simulink model "IEEE33_TR_TEMPORAL_RECOGNIZABILITY_MASTER"  (R2026b)
settings: Solver=ode23t  StopTime=0.2  MaxStep=1e-5
undefined symbols (not defined in the file): Three_PhaseBreaker_class, Three_PhaseSeriesRLCLoad_class, Three_PhaseSource_class, Three_PhaseV_IMeasuremen_class
libraries: ee_lib x146, nesl_utility x106, fl_lib x33, eeRmsMeasurement x2
(part 2 of 7)

== system IEEE33_TR_TEMPORAL_RECOGNIZABILITY_MASTER/Bus_22 ==
  Bus Load 22 : Subsystem
      settings: AttributesFormatString=\n  OpenFcn=elec.conv.unmask(gcb);
  Bus_22 : Subsystem
      settings: OpenFcn=elec.conv.unmask(gcb);
  CB3-2 : Subsystem
      settings: OpenFcn=elec.conv.unmask(gcb);
  VI Recorder3 : Subsystem
  InPhaseA : PMIOPort  Side=Left
  InPhaseB : PMIOPort  Port=2  Side=Left
  InPhaseC : PMIOPort  Port=3  Side=Left
  OutPhaseA : PMIOPort  Port=4  Side=Right
  OutPhaseB : PMIOPort  Port=5  Side=Right
  OutPhaseC : PMIOPort  Port=6  Side=Right
  wires:
  [CB22to12] -> CB3-2/1(com)
  Bus_22/2(Iabc) -> VI Recorder3/2(Irec)
  Bus_22/1(Vabc) -> VI Recorder3/1(Vrec)
  connections:
  CB3-2/RConn3 -- OutPhaseC/RConn1
  Bus_22/RConn2 -- Bus Load 22/LConn2 -- CB3-2/LConn2
  Bus_22/RConn3 -- Bus Load 22/LConn3 -- CB3-2/LConn3
  CB3-2/RConn1 -- OutPhaseA/RConn1
  CB3-2/RConn2 -- OutPhaseB/RConn1
  Bus Load 22/LConn1 -- CB3-2/LConn1 -- Bus_22/RConn1
  InPhaseA/RConn1 -- Bus_22/LConn1
  InPhaseB/RConn1 -- Bus_22/LConn2
  InPhaseC/RConn1 -- Bus_22/LConn3

== system IEEE33_TR_TEMPORAL_RECOGNIZABILITY_MASTER/Bus_23 ==
  Bus Load 23 : Subsystem
      settings: AttributesFormatString=\n  OpenFcn=elec.conv.unmask(gcb);
  Bus_23 : Subsystem
      settings: OpenFcn=elec.conv.unmask(gcb);
  CB3-2 : Subsystem
      settings: OpenFcn=elec.conv.unmask(gcb);
  VI Recorder32 : Subsystem
  InPhaseA : PMIOPort  Side=Left
  InPhaseB : PMIOPort  Port=2  Side=Left
  InPhaseC : PMIOPort  Port=3  Side=Left
  OutPhaseA : PMIOPort  Port=4  Side=Right
  OutPhaseB : PMIOPort  Port=5  Side=Right
  OutPhaseC : PMIOPort  Port=6  Side=Right
  wires:
  Bus_23/2(Iabc) -> VI Recorder32/2(Irec)
  Bus_23/1(Vabc) -> VI Recorder32/1(Vrec)
  [CB23to24] -> CB3-2/1(com)
  connections:
  Bus_23/RConn1 -- CB3-2/LConn1 -- Bus Load 23/LConn1
  CB3-2/RConn3 -- OutPhaseC/RConn1
  Bus Load 23/LConn2 -- CB3-2/LConn2 -- Bus_23/RConn2
  Bus Load 23/LConn3 -- CB3-2/LConn3 -- Bus_23/RConn3
  CB3-2/RConn1 -- OutPhaseA/RConn1
  CB3-2/RConn2 -- OutPhaseB/RConn1
  InPhaseA/RConn1 -- Bus_23/LConn1
  InPhaseB/RConn1 -- Bus_23/LConn2
  InPhaseC/RConn1 -- Bus_23/LConn3

== system IEEE33_TR_TEMPORAL_RECOGNIZABILITY_MASTER/Bus_24 ==
  Bus Load 24 : Subsystem
      settings: AttributesFormatString=\n  OpenFcn=elec.conv.unmask(gcb);
  Bus_24 : Subsystem
      settings: OpenFcn=elec.conv.unmask(gcb);
  CB3-2 : Subsystem
      settings: OpenFcn=elec.conv.unmask(gcb);
  VI Recorder31 : Subsystem
  InPhaseA : PMIOPort  Side=Left
  InPhaseB : PMIOPort  Port=2  Side=Left
  InPhaseC : PMIOPort  Port=3  Side=Left
  OutPhaseA : PMIOPort  Port=4  Side=Right
  OutPhaseB : PMIOPort  Port=5  Side=Right
  OutPhaseC : PMIOPort  Port=6  Side=Right
  wires:
  Bus_24/1(Vabc) -> VI Recorder31/1(Vrec)
  Bus_24/2(Iabc) -> VI Recorder31/2(Irec)
  [CB24to25] -> CB3-2/1(com)
  connections:
  Bus_24/RConn1 -- CB3-2/LConn1 -- Bus Load 24/LConn1
  CB3-2/RConn3 -- OutPhaseC/RConn1
  Bus Load 24/LConn2 -- CB3-2/LConn2 -- Bus_24/RConn2
  Bus Load 24/LConn3 -- CB3-2/LConn3 -- Bus_24/RConn3
  CB3-2/RConn1 -- OutPhaseA/RConn1
  CB3-2/RConn2 -- OutPhaseB/RConn1
  InPhaseA/RConn1 -- Bus_24/LConn1
  InPhaseB/RConn1 -- Bus_24/LConn2
  InPhaseC/RConn1 -- Bus_24/LConn3

== system IEEE33_TR_TEMPORAL_RECOGNIZABILITY_MASTER/Bus_25 ==
  Bus Load 25 : Subsystem
      settings: AttributesFormatString=\n  OpenFcn=elec.conv.unmask(gcb);
  Bus_25 : Subsystem
      settings: OpenFcn=elec.conv.unmask(gcb);
  CB3-2 : Subsystem
      settings: OpenFcn=elec.conv.unmask(gcb);
  VI Recorder30 : Subsystem
  InPhaseA : PMIOPort  Side=Left
  InPhaseB : PMIOPort  Port=2  Side=Left
  InPhaseC : PMIOPort  Port=3  Side=Left
  OutPhaseA : PMIOPort  Port=4  Side=Right
  OutPhaseB : PMIOPort  Port=5  Side=Right
  OutPhaseC : PMIOPort  Port=6  Side=Right
  wires:
  Bus_25/2(Iabc) -> VI Recorder30/2(Irec)
  Bus_25/1(Vabc) -> VI Recorder30/1(Vrec)
  [CB25to29] -> CB3-2/1(com)
  connections:
  Bus_25/RConn1 -- CB3-2/LConn1 -- Bus Load 25/LConn1
  CB3-2/RConn3 -- OutPhaseC/RConn1
  Bus Load 25/LConn2 -- CB3-2/LConn2 -- Bus_25/RConn2
  Bus_25/RConn3 -- CB3-2/LConn3 -- Bus Load 25/LConn3
  CB3-2/RConn1 -- OutPhaseA/RConn1
  CB3-2/RConn2 -- OutPhaseB/RConn1
  InPhaseB/RConn1 -- Bus_25/LConn2
  InPhaseA/RConn1 -- Bus_25/LConn1
  InPhaseC/RConn1 -- Bus_25/LConn3

== system IEEE33_TR_TEMPORAL_RECOGNIZABILITY_MASTER/Bus_26 ==
  Bus Load 26 : Subsystem
      settings: AttributesFormatString=\n  OpenFcn=elec.conv.unmask(gcb);
  Bus_26 : Subsystem
      settings: OpenFcn=elec.conv.unmask(gcb);
  CB3-2 : Subsystem
      settings: OpenFcn=elec.conv.unmask(gcb);
  VI Recorder22 : Subsystem
  InPhaseA : PMIOPort  Side=Left
  InPhaseB : PMIOPort  Port=2  Side=Left
  InPhaseC : PMIOPort  Port=3  Side=Left
  OutPhaseA : PMIOPort  Port=4  Side=Right
  OutPhaseB : PMIOPort  Port=5  Side=Right
  OutPhaseC : PMIOPort  Port=6  Side=Right
  wires:
  Bus_26/2(Iabc) -> VI Recorder22/2(Irec)
  Bus_26/1(Vabc) -> VI Recorder22/1(Vrec)
  [CB26to27] -> CB3-2/1(com)
  connections:
  CB3-2/RConn3 -- OutPhaseC/RConn1
  Bus Load 26/LConn2 -- CB3-2/LConn2 -- Bus_26/RConn2
  Bus_26/RConn3 -- CB3-2/LConn3 -- Bus Load 26/LConn3
  CB3-2/RConn1 -- OutPhaseA/RConn1
  CB3-2/RConn2 -- OutPhaseB/RConn1
  Bus_26/RConn1 -- CB3-2/LConn1 -- Bus Load 26/LConn1
  InPhaseA/RConn1 -- Bus_26/LConn1
  InPhaseB/RConn1 -- Bus_26/LConn2
  InPhaseC/RConn1 -- Bus_26/LConn3

== system IEEE33_TR_TEMPORAL_RECOGNIZABILITY_MASTER/Bus_27 ==
  Bus Load 27 : Subsystem
      settings: AttributesFormatString=\n  OpenFcn=elec.conv.unmask(gcb);
  Bus_27 : Subsystem
      settings: OpenFcn=elec.conv.unmask(gcb);
  CB3-2 : Subsystem
      settings: OpenFcn=elec.conv.unmask(gcb);
  VI Recorder23 : Subsystem
  InPhaseA : PMIOPort  Side=Left
  InPhaseB : PMIOPort  Port=2  Side=Left
  InPhaseC : PMIOPort  Port=3  Side=Left
  OutPhaseA : PMIOPort  Port=4  Side=Right
  OutPhaseB : PMIOPort  Port=5  Side=Right
  OutPhaseC : PMIOPort  Port=6  Side=Right
  wires:
  Bus_27/1(Vabc) -> VI Recorder23/1(Vrec)
  Bus_27/2(Iabc) -> VI Recorder23/2(Irec)
  [CB27to28] -> CB3-2/1(com)
  connections:
  CB3-2/LConn1 -- Bus Load 27/LConn1 -- Bus_27/RConn1
  CB3-2/RConn3 -- OutPhaseC/RConn1
  CB3-2/LConn2 -- Bus Load 27/LConn2 -- Bus_27/RConn2
  Bus_27/RConn3 -- Bus Load 27/LConn3 -- CB3-2/LConn3
  CB3-2/RConn1 -- OutPhaseA/RConn1
  CB3-2/RConn2 -- OutPhaseB/RConn1
  InPhaseA/RConn1 -- Bus_27/LConn1
  InPhaseB/RConn1 -- Bus_27/LConn2
  InPhaseC/RConn1 -- Bus_27/LConn3

== system IEEE33_TR_TEMPORAL_RECOGNIZABILITY_MASTER/Bus_28 ==
  Bus Load 28 : Subsystem
      settings: AttributesFormatString=\n  OpenFcn=elec.conv.unmask(gcb);
  Bus_28 : Subsystem
      settings: OpenFcn=elec.conv.unmask(gcb);
  CB3-2 : Subsystem
      settings: OpenFcn=elec.conv.unmask(gcb);
  VI Recorder24 : Subsystem
  InPhaseA : PMIOPort  Side=Left
  InPhaseB : PMIOPort  Port=2  Side=Left
  InPhaseC : PMIOPort  Port=3  Side=Left
  OutPhaseA : PMIOPort  Port=4  Side=Right
  OutPhaseB : PMIOPort  Port=5  Side=Right
  OutPhaseC : PMIOPort  Port=6  Side=Right
  wires:
  Bus_28/2(Iabc) -> VI Recorder24/2(Irec)
  Bus_28/1(Vabc) -> VI Recorder24/1(Vrec)
  [CB28to29] -> CB3-2/1(com)
  connections:
  Bus Load 28/LConn1 -- CB3-2/LConn1 -- Bus_28/RConn1
  CB3-2/RConn3 -- OutPhaseC/RConn1
  Bus Load 28/LConn2 -- CB3-2/LConn2 -- Bus_28/RConn2
  Bus Load 28/LConn3 -- CB3-2/LConn3 -- Bus_28/RConn3
  CB3-2/RConn1 -- OutPhaseA/RConn1
  CB3-2/RConn2 -- OutPhaseB/RConn1
  InPhaseA/RConn1 -- Bus_28/LConn1
  InPhaseB/RConn1 -- Bus_28/LConn2
  InPhaseC/RConn1 -- Bus_28/LConn3

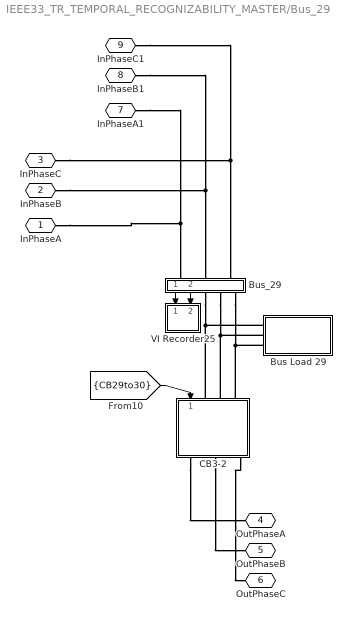
== system IEEE33_TR_TEMPORAL_RECOGNIZABILITY_MASTER/Bus_29 ==
  Bus Load 29 : Subsystem
      settings: AttributesFormatString=\n  OpenFcn=elec.conv.unmask(gcb);
  Bus_29 : Subsystem
      settings: OpenFcn=elec.conv.unmask(gcb);
  CB3-2 : Subsystem
      settings: OpenFcn=elec.conv.unmask(gcb);
  VI Recorder25 : Subsystem
  InPhaseA : PMIOPort  Side=Left
  InPhaseB : PMIOPort  Port=2  Side=Left
  InPhaseC : PMIOPort  Port=3  Side=Left
  OutPhaseA : PMIOPort  Port=4  Side=Right
  OutPhaseB : PMIOPort  Port=5  Side=Right
  OutPhaseC : PMIOPort  Port=6  Side=Right
  InPhaseA1 : PMIOPort  Port=7  Side=Left
  InPhaseB1 : PMIOPort  Port=8  Side=Left
  InPhaseC1 : PMIOPort  Port=9  Side=Left
  wires:
  Bus_29/1(Vabc) -> VI Recorder25/1(Vrec)
  Bus_29/2(Iabc) -> VI Recorder25/2(Irec)
  [CB29to30] -> CB3-2/1(com)
  connections:
  Bus_29/RConn1 -- CB3-2/LConn1 -- Bus Load 29/LConn1
  CB3-2/RConn3 -- OutPhaseC/RConn1
  Bus Load 29/LConn2 -- CB3-2/LConn2 -- Bus_29/RConn2
  Bus Load 29/LConn3 -- CB3-2/LConn3 -- Bus_29/RConn3
  CB3-2/RConn1 -- OutPhaseA/RConn1
  CB3-2/RConn2 -- OutPhaseB/RConn1
  InPhaseB1/RConn1 -- InPhaseB/RConn1 -- Bus_29/LConn2
  InPhaseA1/RConn1 -- InPhaseA/RConn1 -- Bus_29/LConn1
  InPhaseC1/RConn1 -- InPhaseC/RConn1 -- Bus_29/LConn3

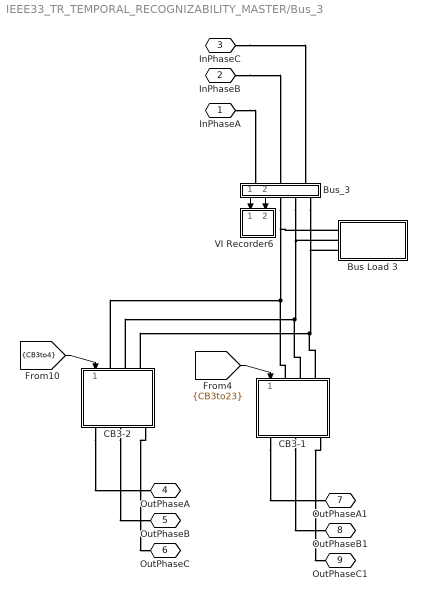
== system IEEE33_TR_TEMPORAL_RECOGNIZABILITY_MASTER/Bus_3 ==
  Bus Load 3 : Subsystem
      settings: AttributesFormatString=\n  OpenFcn=elec.conv.unmask(gcb);
  Bus_3 : Subsystem
      settings: OpenFcn=elec.conv.unmask(gcb);
  CB3-1 : Subsystem
      settings: OpenFcn=elec.conv.unmask(gcb);
  CB3-2 : Subsystem
      settings: OpenFcn=elec.conv.unmask(gcb);
  VI Recorder6 : Subsystem
  InPhaseA : PMIOPort  Side=Left
  InPhaseB : PMIOPort  Port=2  Side=Left
  InPhaseC : PMIOPort  Port=3  Side=Left
  OutPhaseA : PMIOPort  Port=4  Side=Right
  OutPhaseB : PMIOPort  Port=5  Side=Right
  OutPhaseC : PMIOPort  Port=6  Side=Right
  OutPhaseA1 : PMIOPort  Port=7  Side=Right
  OutPhaseB1 : PMIOPort  Port=8  Side=Right
  OutPhaseC1 : PMIOPort  Port=9  Side=Right
  wires:
  Bus_3/2(Iabc) -> VI Recorder6/2(Irec)
  Bus_3/1(Vabc) -> VI Recorder6/1(Vrec)
  [CB3to4] -> CB3-2/1(com)
  [CB3to23] -> CB3-1/1(com)
  connections:
  CB3-2/LConn1 -- CB3-1/LConn1 -- Bus Load 3/LConn1 -- Bus_3/RConn1
  CB3-2/RConn3 -- OutPhaseC/RConn1
  CB3-1/LConn2 -- Bus Load 3/LConn2 -- Bus_3/RConn2 -- CB3-2/LConn2
  CB3-1/LConn3 -- Bus_3/RConn3 -- Bus Load 3/LConn3 -- CB3-2/LConn3
  CB3-2/RConn1 -- OutPhaseA/RConn1
  CB3-2/RConn2 -- OutPhaseB/RConn1
  CB3-1/RConn3 -- OutPhaseC1/RConn1
  CB3-1/RConn1 -- OutPhaseA1/RConn1
  CB3-1/RConn2 -- OutPhaseB1/RConn1
  InPhaseA/RConn1 -- Bus_3/LConn1
  InPhaseB/RConn1 -- Bus_3/LConn2
  InPhaseC/RConn1 -- Bus_3/LConn3

== system IEEE33_TR_TEMPORAL_RECOGNIZABILITY_MASTER/Bus_30 ==
  Bus Load 30 : Subsystem
      settings: AttributesFormatString=\n  OpenFcn=elec.conv.unmask(gcb);
  Bus_30 : Subsystem
      settings: OpenFcn=elec.conv.unmask(gcb);
  CB3-2 : Subsystem
      settings: OpenFcn=elec.conv.unmask(gcb);
  VI Recorder26 : Subsystem
  InPhaseA : PMIOPort  Side=Left
  InPhaseB : PMIOPort  Port=2  Side=Left
  InPhaseC : PMIOPort  Port=3  Side=Left
  OutPhaseA : PMIOPort  Port=4  Side=Right
  OutPhaseB : PMIOPort  Port=5  Side=Right
  OutPhaseC : PMIOPort  Port=6  Side=Right
  wires:
  Bus_30/1(Vabc) -> VI Recorder26/1(Vrec)
  Bus_30/2(Iabc) -> VI Recorder26/2(Irec)
  [CB30to31] -> CB3-2/1(com)
  connections:
  Bus_30/RConn1 -- CB3-2/LConn1 -- Bus Load 30/LConn1
  CB3-2/RConn3 -- OutPhaseC/RConn1
  Bus Load 30/LConn2 -- CB3-2/LConn2 -- Bus_30/RConn2
  Bus Load 30/LConn3 -- CB3-2/LConn3 -- Bus_30/RConn3
  CB3-2/RConn1 -- OutPhaseA/RConn1
  CB3-2/RConn2 -- OutPhaseB/RConn1
  InPhaseB/RConn1 -- Bus_30/LConn2
  InPhaseA/RConn1 -- Bus_30/LConn1
  InPhaseC/RConn1 -- Bus_30/LConn3

== system IEEE33_TR_TEMPORAL_RECOGNIZABILITY_MASTER/Bus_31 ==
  Bus Load 31 : Subsystem
      settings: AttributesFormatString=\n  OpenFcn=elec.conv.unmask(gcb);
  Bus_31 : Subsystem
      settings: OpenFcn=elec.conv.unmask(gcb);
  CB3-2 : Subsystem
      settings: OpenFcn=elec.conv.unmask(gcb);
  VI Recorder27 : Subsystem
  InPhaseA : PMIOPort  Side=Left
  InPhaseB : PMIOPort  Port=2  Side=Left
  InPhaseC : PMIOPort  Port=3  Side=Left
  OutPhaseA : PMIOPort  Port=4  Side=Right
  OutPhaseB : PMIOPort  Port=5  Side=Right
  OutPhaseC : PMIOPort  Port=6  Side=Right
  wires:
  Bus_31/2(Iabc) -> VI Recorder27/2(Irec)
  Bus_31/1(Vabc) -> VI Recorder27/1(Vrec)
  [CB31to32] -> CB3-2/1(com)
  connections:
  Bus_31/RConn1 -- CB3-2/LConn1 -- Bus Load 31/LConn1
  CB3-2/RConn3 -- OutPhaseC/RConn1
  Bus Load 31/LConn2 -- CB3-2/LConn2 -- Bus_31/RConn2
  Bus Load 31/LConn3 -- CB3-2/LConn3 -- Bus_31/RConn3
  CB3-2/RConn1 -- OutPhaseA/RConn1
  CB3-2/RConn2 -- OutPhaseB/RConn1
  InPhaseA/RConn1 -- Bus_31/LConn1
  Bus_31/LConn2 -- InPhaseB/RConn1
  InPhaseC/RConn1 -- Bus_31/LConn3

== system IEEE33_TR_TEMPORAL_RECOGNIZABILITY_MASTER/Bus_32 ==
  Bus Load 32 : Subsystem
      settings: AttributesFormatString=\n  OpenFcn=elec.conv.unmask(gcb);
  Bus_32 : Subsystem
      settings: OpenFcn=elec.conv.unmask(gcb);
  CB3-2 : Subsystem
      settings: OpenFcn=elec.conv.unmask(gcb);
  VI Recorder28 : Subsystem
  InPhaseA : PMIOPort  Side=Left
  InPhaseB : PMIOPort  Port=2  Side=Left
  InPhaseC : PMIOPort  Port=3  Side=Left
  OutPhaseA : PMIOPort  Port=4  Side=Right
  OutPhaseB : PMIOPort  Port=5  Side=Right
  OutPhaseC : PMIOPort  Port=6  Side=Right
  wires:
  Bus_32/2(Iabc) -> VI Recorder28/2(Irec)
  Bus_32/1(Vabc) -> VI Recorder28/1(Vrec)
  [CB32to33] -> CB3-2/1(com)
  connections:
  Bus_32/RConn1 -- CB3-2/LConn1 -- Bus Load 32/LConn1
  CB3-2/RConn3 -- OutPhaseC/RConn1
  Bus Load 32/LConn2 -- CB3-2/LConn2 -- Bus_32/RConn2
  Bus_32/RConn3 -- Bus Load 32/LConn3 -- CB3-2/LConn3
  CB3-2/RConn1 -- OutPhaseA/RConn1
  CB3-2/RConn2 -- OutPhaseB/RConn1
  InPhaseA/RConn1 -- Bus_32/LConn1
  InPhaseB/RConn1 -- Bus_32/LConn2
  InPhaseC/RConn1 -- Bus_32/LConn3

== system IEEE33_TR_TEMPORAL_RECOGNIZABILITY_MASTER/Bus_33 ==
  Bus Load 33 : Subsystem
      settings: AttributesFormatString=\n  OpenFcn=elec.conv.unmask(gcb);
  Bus_33 : Subsystem
      settings: OpenFcn=elec.conv.unmask(gcb);
  VI Recorder29 : Subsystem
  InPhaseA : PMIOPort  Side=Left
  InPhaseB : PMIOPort  Port=2  Side=Left
  InPhaseC : PMIOPort  Port=3  Side=Left
  OutPhaseA : PMIOPort  Port=4  Side=Right
  OutPhaseB : PMIOPort  Port=5  Side=Right
  OutPhaseC : PMIOPort  Port=6  Side=Right
  wires:
  Bus_33/2(Iabc) -> VI Recorder29/2(Irec)
  Bus_33/1(Vabc) -> VI Recorder29/1(Vrec)
  connections:
  Bus Load 33/LConn1 -- Bus_33/RConn1 -- OutPhaseA/RConn1
  Bus Load 33/LConn2 -- OutPhaseB/RConn1 -- Bus_33/RConn2
  Bus_33/RConn3 -- OutPhaseC/RConn1 -- Bus Load 33/LConn3
  InPhaseA/RConn1 -- Bus_33/LConn1
  InPhaseB/RConn1 -- Bus_33/LConn2
  InPhaseC/RConn1 -- Bus_33/LConn3

== system IEEE33_TR_TEMPORAL_RECOGNIZABILITY_MASTER/Bus_4 ==
  Bus Load 4 : Subsystem
      settings: AttributesFormatString=\n  OpenFcn=elec.conv.unmask(gcb);
  Bus_4 : Subsystem
      settings: OpenFcn=elec.conv.unmask(gcb);
  CB3-2 : Subsystem
      settings: OpenFcn=elec.conv.unmask(gcb);
  VI Recorder7 : Subsystem
  InPhaseA : PMIOPort  Side=Left
  InPhaseB : PMIOPort  Port=2  Side=Left
  InPhaseC : PMIOPort  Port=3  Side=Left
  OutPhaseA : PMIOPort  Port=4  Side=Right
  OutPhaseB : PMIOPort  Port=5  Side=Right
  OutPhaseC : PMIOPort  Port=6  Side=Right
  wires:
  Bus_4/1(Vabc) -> VI Recorder7/1(Vrec)
  Bus_4/2(Iabc) -> VI Recorder7/2(Irec)
  [CB4to5] -> CB3-2/1(com)
  connections:
  Bus_4/RConn1 -- CB3-2/LConn1 -- Bus Load 4/LConn1
  CB3-2/RConn3 -- OutPhaseC/RConn1
  Bus Load 4/LConn2 -- CB3-2/LConn2 -- Bus_4/RConn2
  Bus_4/RConn3 -- CB3-2/LConn3 -- Bus Load 4/LConn3
  CB3-2/RConn1 -- OutPhaseA/RConn1
  CB3-2/RConn2 -- OutPhaseB/RConn1
  InPhaseA/RConn1 -- Bus_4/LConn1
  InPhaseB/RConn1 -- Bus_4/LConn2
  InPhaseC/RConn1 -- Bus_4/LConn3

== system IEEE33_TR_TEMPORAL_RECOGNIZABILITY_MASTER/Bus_5 ==
  Bus Load 5 : Subsystem
      settings: AttributesFormatString=\n  OpenFcn=elec.conv.unmask(gcb);
  Bus_5 : Subsystem
      settings: OpenFcn=elec.conv.unmask(gcb);
  CB3-2 : Subsystem
      settings: OpenFcn=elec.conv.unmask(gcb);
  VI Recorder8 : Subsystem
  InPhaseA : PMIOPort  Side=Left
  InPhaseB : PMIOPort  Port=2  Side=Left
  InPhaseC : PMIOPort  Port=3  Side=Left
  OutPhaseA : PMIOPort  Port=4  Side=Right
  OutPhaseB : PMIOPort  Port=5  Side=Right
  OutPhaseC : PMIOPort  Port=6  Side=Right
  wires:
  Bus_5/2(Iabc) -> VI Recorder8/2(Irec)
  Bus_5/1(Vabc) -> VI Recorder8/1(Vrec)
  [CB5to6] -> CB3-2/1(com)
  connections:
  Bus Load 5/LConn1 -- CB3-2/LConn1 -- Bus_5/RConn1
  CB3-2/RConn3 -- OutPhaseC/RConn1
  Bus_5/RConn2 -- CB3-2/LConn2 -- Bus Load 5/LConn2
  Bus_5/RConn3 -- CB3-2/LConn3 -- Bus Load 5/LConn3
  CB3-2/RConn1 -- OutPhaseA/RConn1
  CB3-2/RConn2 -- OutPhaseB/RConn1
  InPhaseA/RConn1 -- Bus_5/LConn1
  InPhaseB/RConn1 -- Bus_5/LConn2
  InPhaseC/RConn1 -- Bus_5/LConn3

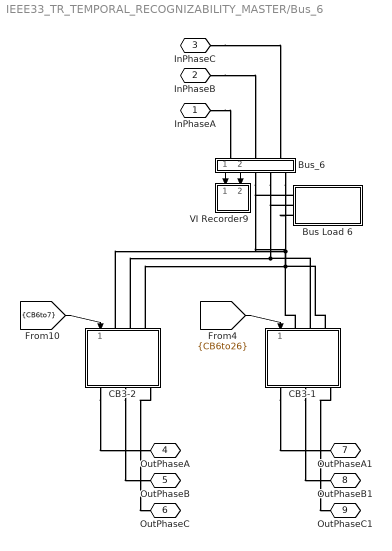
== system IEEE33_TR_TEMPORAL_RECOGNIZABILITY_MASTER/Bus_6 ==
  Bus Load 6 : Subsystem
      settings: AttributesFormatString=\n  OpenFcn=elec.conv.unmask(gcb);
  Bus_6 : Subsystem
      settings: OpenFcn=elec.conv.unmask(gcb);
  CB3-1 : Subsystem
      settings: OpenFcn=elec.conv.unmask(gcb);
  CB3-2 : Subsystem
      settings: OpenFcn=elec.conv.unmask(gcb);
  VI Recorder9 : Subsystem
  InPhaseA : PMIOPort  Side=Left
  InPhaseB : PMIOPort  Port=2  Side=Left
  InPhaseC : PMIOPort  Port=3  Side=Left
  OutPhaseA : PMIOPort  Port=4  Side=Right
  OutPhaseB : PMIOPort  Port=5  Side=Right
  OutPhaseC : PMIOPort  Port=6  Side=Right
  OutPhaseA1 : PMIOPort  Port=7  Side=Right
  OutPhaseB1 : PMIOPort  Port=8  Side=Right
  OutPhaseC1 : PMIOPort  Port=9  Side=Right
  wires:
  Bus_6/1(Vabc) -> VI Recorder9/1(Vrec)
  Bus_6/2(Iabc) -> VI Recorder9/2(Irec)
  [CB6to26] -> CB3-1/1(com)
  [CB6to7] -> CB3-2/1(com)
  connections:
  Bus Load 6/LConn1 -- Bus_6/RConn1 -- CB3-2/LConn1 -- CB3-1/LConn1
  CB3-2/RConn3 -- OutPhaseC/RConn1
  Bus Load 6/LConn2 -- Bus_6/RConn2 -- CB3-1/LConn2 -- CB3-2/LConn2
  Bus Load 6/LConn3 -- Bus_6/RConn3 -- CB3-1/LConn3 -- CB3-2/LConn3
  CB3-2/RConn1 -- OutPhaseA/RConn1
  CB3-2/RConn2 -- OutPhaseB/RConn1
  CB3-1/RConn3 -- OutPhaseC1/RConn1
  CB3-1/RConn2 -- OutPhaseB1/RConn1
  CB3-1/RConn1 -- OutPhaseA1/RConn1
  InPhaseA/RConn1 -- Bus_6/LConn1
  InPhaseB/RConn1 -- Bus_6/LConn2
  InPhaseC/RConn1 -- Bus_6/LConn3

== system IEEE33_TR_TEMPORAL_RECOGNIZABILITY_MASTER/Bus_7 ==
  Bus Load 7 : Subsystem
      settings: AttributesFormatString=\n  OpenFcn=elec.conv.unmask(gcb);
  Bus_7 : Subsystem
      settings: OpenFcn=elec.conv.unmask(gcb);
  CB3-2 : Subsystem
      settings: OpenFcn=elec.conv.unmask(gcb);
  VI Recorder10 : Subsystem
  InPhaseA : PMIOPort  Side=Left
  InPhaseB : PMIOPort  Port=2  Side=Left
  InPhaseC : PMIOPort  Port=3  Side=Left
  OutPhaseA : PMIOPort  Port=4  Side=Right
  OutPhaseB : PMIOPort  Port=5  Side=Right
  OutPhaseC : PMIOPort  Port=6  Side=Right
  wires:
  Bus_7/2(Iabc) -> VI Recorder10/2(Irec)
  Bus_7/1(Vabc) -> VI Recorder10/1(Vrec)
  [CB7to8] -> CB3-2/1(com)
  connections:
  Bus_7/RConn1 -- CB3-2/LConn1 -- Bus Load 7/LConn1
  CB3-2/RConn3 -- OutPhaseC/RConn1
  Bus Load 7/LConn2 -- CB3-2/LConn2 -- Bus_7/RConn2
  CB3-2/LConn3 -- Bus Load 7/LConn3 -- Bus_7/RConn3
  CB3-2/RConn1 -- OutPhaseA/RConn1
  CB3-2/RConn2 -- OutPhaseB/RConn1
  InPhaseA/RConn1 -- Bus_7/LConn1
  InPhaseB/RConn1 -- Bus_7/LConn2
  InPhaseC/RConn1 -- Bus_7/LConn3

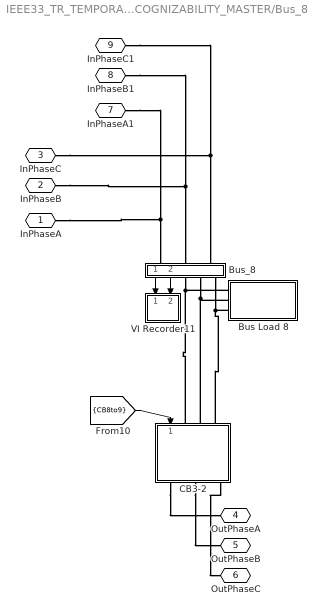
== system IEEE33_TR_TEMPORAL_RECOGNIZABILITY_MASTER/Bus_8 ==
  Bus Load 8 : Subsystem
      settings: AttributesFormatString=\n  OpenFcn=elec.conv.unmask(gcb);
  Bus_8 : Subsystem
      settings: OpenFcn=elec.conv.unmask(gcb);
  CB3-2 : Subsystem
      settings: OpenFcn=elec.conv.unmask(gcb);
  VI Recorder11 : Subsystem
  InPhaseA : PMIOPort  Side=Left
  InPhaseB : PMIOPort  Port=2  Side=Left
  InPhaseC : PMIOPort  Port=3  Side=Left
  OutPhaseA : PMIOPort  Port=4  Side=Right
  OutPhaseB : PMIOPort  Port=5  Side=Right
  OutPhaseC : PMIOPort  Port=6  Side=Right
  InPhaseA1 : PMIOPort  Port=7  Side=Left
  InPhaseB1 : PMIOPort  Port=8  Side=Left
  InPhaseC1 : PMIOPort  Port=9  Side=Left
  wires:
  Bus_8/2(Iabc) -> VI Recorder11/2(Irec)
  Bus_8/1(Vabc) -> VI Recorder11/1(Vrec)
  [CB8to9] -> CB3-2/1(com)
  connections:
  Bus Load 8/LConn1 -- CB3-2/LConn1 -- Bus_8/RConn1
  CB3-2/RConn3 -- OutPhaseC/RConn1
  Bus Load 8/LConn2 -- CB3-2/LConn2 -- Bus_8/RConn2
  Bus_8/RConn3 -- CB3-2/LConn3 -- Bus Load 8/LConn3
  CB3-2/RConn1 -- OutPhaseA/RConn1
  CB3-2/RConn2 -- OutPhaseB/RConn1
  InPhaseA1/RConn1 -- InPhaseA/RConn1 -- Bus_8/LConn1
  InPhaseB1/RConn1 -- InPhaseB/RConn1 -- Bus_8/LConn2
  InPhaseC1/RConn1 -- InPhaseC/RConn1 -- Bus_8/LConn3

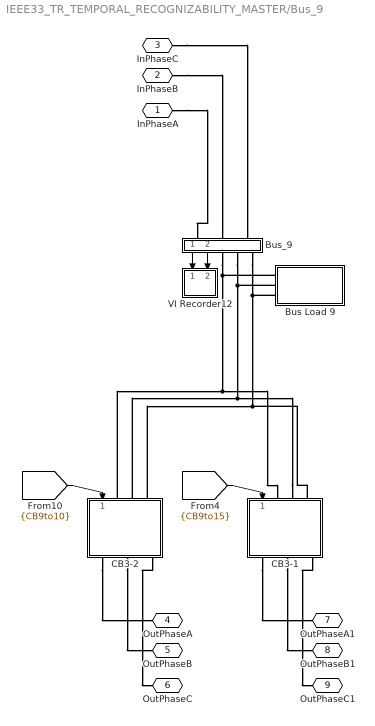
== system IEEE33_TR_TEMPORAL_RECOGNIZABILITY_MASTER/Bus_9 ==
  Bus Load 9 : Subsystem
      settings: AttributesFormatString=\n  OpenFcn=elec.conv.unmask(gcb);
  Bus_9 : Subsystem
      settings: OpenFcn=elec.conv.unmask(gcb);
  CB3-1 : Subsystem
      settings: OpenFcn=elec.conv.unmask(gcb);
  CB3-2 : Subsystem
      settings: OpenFcn=elec.conv.unmask(gcb);
  VI Recorder12 : Subsystem
  InPhaseA : PMIOPort  Side=Left
  InPhaseB : PMIOPort  Port=2  Side=Left
  InPhaseC : PMIOPort  Port=3  Side=Left
  OutPhaseA : PMIOPort  Port=4  Side=Right
  OutPhaseB : PMIOPort  Port=5  Side=Right
  OutPhaseC : PMIOPort  Port=6  Side=Right
  OutPhaseA1 : PMIOPort  Port=7  Side=Right
  OutPhaseB1 : PMIOPort  Port=8  Side=Right
  OutPhaseC1 : PMIOPort  Port=9  Side=Right
  wires:
  Bus_9/2(Iabc) -> VI Recorder12/2(Irec)
  Bus_9/1(Vabc) -> VI Recorder12/1(Vrec)
  [CB9to10] -> CB3-2/1(com)
  [CB9to15] -> CB3-1/1(com)
  connections:
  CB3-1/LConn1 -- Bus Load 9/LConn1 -- Bus_9/RConn1 -- CB3-2/LConn1
  CB3-2/RConn3 -- OutPhaseC/RConn1
  CB3-1/LConn2 -- Bus_9/RConn2 -- Bus Load 9/LConn2 -- CB3-2/LConn2
  Bus Load 9/LConn3 -- Bus_9/RConn3 -- CB3-1/LConn3 -- CB3-2/LConn3
  CB3-2/RConn1 -- OutPhaseA/RConn1
  CB3-2/RConn2 -- OutPhaseB/RConn1
  InPhaseA/RConn1 -- Bus_9/LConn1
  InPhaseB/RConn1 -- Bus_9/LConn2
  InPhaseC/RConn1 -- Bus_9/LConn3
  CB3-1/RConn2 -- OutPhaseB1/RConn1
  CB3-1/RConn3 -- OutPhaseC1/RConn1
  CB3-1/RConn1 -- OutPhaseA1/RConn1

== system IEEE33_TR_TEMPORAL_RECOGNIZABILITY_MASTER/Incoming1 ==
  Electrical Reference : fl_lib/Electrical/Electrical Elements/Electrical Reference
  Voltage Source : ee_lib/Sources/Voltage Source (Three-Phase)  vline_rms=12660 V  shift=0 deg  freq=60 Hz  impedance_option=0  SShortCircuit=438555000 V*A  XR=7  R=Three_PhaseSource_class(12660,50,0.8929,0.01658,438555000,12660,7,'off','on').objParamMappingDerived.NewDerivedParam.R Ohm  L=Three_PhaseSource_class(12660,50,0.8929,0.01658,438555000,12660,7,'off','on').objParamMappingDerived.NewDerivedParam.L H  harmonic_option=0  harmonic_orders=[5, 7, 11, 13]  harmonic_ratios=[.1, .1, .1, .1]  G_parasitic=0 1/Ohm  I_specify=off  I_priority=None  I=[ 0 0 0 ] A  I_nominal_specify=off  I_nominal_value=1  I_nominal_unit=A
  A : PMIOPort  Side=Right
  B : PMIOPort  Port=2  Side=Right
  C : PMIOPort  Port=3  Side=Right
  connections:
  Voltage Source/RConn2 -- B/RConn1
  Voltage Source/RConn1 -- A/RConn1
  Voltage Source/RConn3 -- C/RConn1
  Electrical Reference/LConn1 -- Voltage Source/LConn1

== system IEEE33_TR_TEMPORAL_RECOGNIZABILITY_MASTER/RMS ==
  In : Inport
  RMS Measurement : eeRmsMeasurement/RMS Measurement  LabelModeActiveChoice=Total  F=60  SpecifyHarmonics=off  K=[0 1 2]  InitialRMS=0  Ts=0
  RMS : Outport  VectorParamsAs1DForOutWhenUnconnected=off
  wires:
  RMS Measurement/1 -> RMS/1
  In/1 -> RMS Measurement/1

== system IEEE33_TR_TEMPORAL_RECOGNIZABILITY_MASTER/RMS1 ==
  In : Inport
  RMS Measurement : eeRmsMeasurement/RMS Measurement  LabelModeActiveChoice=Total  F=60  SpecifyHarmonics=off  K=[0 1 2]  InitialRMS=0  Ts=0
  RMS : Outport  VectorParamsAs1DForOutWhenUnconnected=off
  wires:
  RMS Measurement/1 -> RMS/1
  In/1 -> RMS Measurement/1

== system IEEE33_TR_TEMPORAL_RECOGNIZABILITY_MASTER/Solver Configuration1 ==
  Solver Configuration : nesl_utility/Solver Configuration  PhysicalDomain=network_engine_domain  SubClassName=solver  LeftPortType=input  RightPortType=generic  Tones=[]  Harmonics=[]  SimulateNoise=off  Profile=off  UseLocalSampling=off  EnableSwitchedLinearOptims=on  FrequencyDomain=off  UseCCode=off  RelTol=0.001  AbsTol=1e-06  MinStep=1e-09  ToWorkspace=off  RevertToSquareIcSolve=off  NumHomotopyIterations=100  PhasorMode=off  PhasorModeNumHarmonics=1  ConsistencySolver=NEWTON_FTOL  CanonicalOrdering=UNORDERED  OptimizeIntermediates=UNOPTIMIZED  MulticoreSolverChoice=BACKWARD_EULER  IndexReductionMethod=DerivativeReplacement  DoDC=off  ResidualTolerance=1e-09  ConsistencyTolSource=GLOBAL  ConsistencyAbsTol=0.001  ConsistencyRelTol=0.001  ConsistencyTolFactor=0.001  UseLocalSolver=on  LocalSolverChoice=NE_BACKWARD_EULER_ADVANCER  ResolveIndetEquations=off  FunctionEvalNumThread=1  LocalSolverSampleTime=1e-05  DoFixedCost=on  MaxNonlinIter=4  MaxModeIter=2  ComputeImpulses=off  ImpulseIterations=1  LinearAlgebra=auto  LinearAlgebraNumThread=0  EquationFormulation=NE_TIME_EF  DelaysMemoryBudget=1024  AutomaticFiltering=on  FilteringTimeConstant=0.001  PartitionStorageMethod=AS_NEEDED  PartitionMemoryBudget=1024  PartitionMethod=FAST  MultibodyUseLocalSolver=off  MultibodyLocalSolverChoice=ODE1  MultibodyLocalSolverSampleTime=0.001
  f(x)=0 : PMIOPort  Side=Right
  connections:
  f(x)=0/RConn1 -- Solver Configuration/RConn1

== system IEEE33_TR_TEMPORAL_RECOGNIZABILITY_MASTER/Three-Phase Series RLC Branch ==
  Three_PhaseSeriesRLCBran : ee_lib/Passive/RLC Assemblies/RLC (Three-Phase)  port_option=ee.enum.threePhasePort.expanded  component_structure=4  R=0.0922 Ohm  L=0.00014961 H  C=1e-06 F  R_parasitic=1e-6 Ohm  G_parasitic=1e-6 1/Ohm  IL_specify=on  IL_priority=High  IL=[0, 0, 0] A  IL_nominal_specify=off  IL_nominal_value=1  IL_nominal_unit=A  VC_specify=on  VC_priority=High  VC=[0, 0, 0] V  VC_nominal_specify=off  VC_nominal_value=1  VC_nominal_unit=V
  A : PMIOPort  Side=Left
  B : PMIOPort  Port=2  Side=Left
  C : PMIOPort  Port=3  Side=Left
  a : PMIOPort  Port=4  Side=Right
  b : PMIOPort  Port=5  Side=Right
  c : PMIOPort  Port=6  Side=Right
  connections:
  Three_PhaseSeriesRLCBran/RConn3 -- c/RConn1
  Three_PhaseSeriesRLCBran/RConn2 -- b/RConn1
  Three_PhaseSeriesRLCBran/RConn1 -- a/RConn1
  C/RConn1 -- Three_PhaseSeriesRLCBran/LConn3
  B/RConn1 -- Three_PhaseSeriesRLCBran/LConn2
  A/RConn1 -- Three_PhaseSeriesRLCBran/LConn1

== system IEEE33_TR_TEMPORAL_RECOGNIZABILITY_MASTER/Three-Phase Series RLC Branch1 ==
  Three_PhaseSeriesRLCBran : ee_lib/Passive/RLC Assemblies/RLC (Three-Phase)  port_option=ee.enum.threePhasePort.expanded  component_structure=4  R=0.493 Ohm  L=0.00079928 H  C=1e-06 F  R_parasitic=1e-6 Ohm  G_parasitic=1e-6 1/Ohm  IL_specify=on  IL_priority=High  IL=[0, 0, 0] A  IL_nominal_specify=off  IL_nominal_value=1  IL_nominal_unit=A  VC_specify=on  VC_priority=High  VC=[0, 0, 0] V  VC_nominal_specify=off  VC_nominal_value=1  VC_nominal_unit=V
  A : PMIOPort  Side=Left
  B : PMIOPort  Port=2  Side=Left
  C : PMIOPort  Port=3  Side=Left
  a : PMIOPort  Port=4  Side=Right
  b : PMIOPort  Port=5  Side=Right
  c : PMIOPort  Port=6  Side=Right
  connections:
  Three_PhaseSeriesRLCBran/RConn3 -- c/RConn1
  Three_PhaseSeriesRLCBran/RConn2 -- b/RConn1
  Three_PhaseSeriesRLCBran/RConn1 -- a/RConn1
  C/RConn1 -- Three_PhaseSeriesRLCBran/LConn3
  B/RConn1 -- Three_PhaseSeriesRLCBran/LConn2
  A/RConn1 -- Three_PhaseSeriesRLCBran/LConn1

== system IEEE33_TR_TEMPORAL_RECOGNIZABILITY_MASTER/Three-Phase Series RLC Branch10 ==
  Three_PhaseSeriesRLCBran : ee_lib/Passive/RLC Assemblies/RLC (Three-Phase)  port_option=ee.enum.threePhasePort.expanded  component_structure=4  R=0.3744 Ohm  L=0.00039407 H  C=1e-06 F  R_parasitic=1e-6 Ohm  G_parasitic=1e-6 1/Ohm  IL_specify=on  IL_priority=High  IL=[0, 0, 0] A  IL_nominal_specify=off  IL_nominal_value=1  IL_nominal_unit=A  VC_specify=on  VC_priority=High  VC=[0, 0, 0] V  VC_nominal_specify=off  VC_nominal_value=1  VC_nominal_unit=V
  A : PMIOPort  Side=Left
  B : PMIOPort  Port=2  Side=Left
  C : PMIOPort  Port=3  Side=Left
  a : PMIOPort  Port=4  Side=Right
  b : PMIOPort  Port=5  Side=Right
  c : PMIOPort  Port=6  Side=Right
  connections:
  Three_PhaseSeriesRLCBran/RConn3 -- c/RConn1
  Three_PhaseSeriesRLCBran/RConn2 -- b/RConn1
  Three_PhaseSeriesRLCBran/RConn1 -- a/RConn1
  C/RConn1 -- Three_PhaseSeriesRLCBran/LConn3
  B/RConn1 -- Three_PhaseSeriesRLCBran/LConn2
  A/RConn1 -- Three_PhaseSeriesRLCBran/LConn1

== system IEEE33_TR_TEMPORAL_RECOGNIZABILITY_MASTER/Three-Phase Series RLC Branch11 ==
  Three_PhaseSeriesRLCBran : ee_lib/Passive/RLC Assemblies/RLC (Three-Phase)  port_option=ee.enum.threePhasePort.expanded  component_structure=4  R=1.468 Ohm  L=0.0036765 H  C=1e-06 F  R_parasitic=1e-6 Ohm  G_parasitic=1e-6 1/Ohm  IL_specify=on  IL_priority=High  IL=[0, 0, 0] A  IL_nominal_specify=off  IL_nominal_value=1  IL_nominal_unit=A  VC_specify=on  VC_priority=High  VC=[0, 0, 0] V  VC_nominal_specify=off  VC_nominal_value=1  VC_nominal_unit=V
  A : PMIOPort  Side=Left
  B : PMIOPort  Port=2  Side=Left
  C : PMIOPort  Port=3  Side=Left
  a : PMIOPort  Port=4  Side=Right
  b : PMIOPort  Port=5  Side=Right
  c : PMIOPort  Port=6  Side=Right
  connections:
  Three_PhaseSeriesRLCBran/RConn3 -- c/RConn1
  Three_PhaseSeriesRLCBran/RConn2 -- b/RConn1
  Three_PhaseSeriesRLCBran/RConn1 -- a/RConn1
  C/RConn1 -- Three_PhaseSeriesRLCBran/LConn3
  B/RConn1 -- Three_PhaseSeriesRLCBran/LConn2
  A/RConn1 -- Three_PhaseSeriesRLCBran/LConn1

== system IEEE33_TR_TEMPORAL_RECOGNIZABILITY_MASTER/Three-Phase Series RLC Branch12 ==
  Three_PhaseSeriesRLCBran : ee_lib/Passive/RLC Assemblies/RLC (Three-Phase)  port_option=ee.enum.threePhasePort.expanded  component_structure=4  R=0.5416 Ohm  L=0.0022692 H  C=1e-06 F  R_parasitic=1e-6 Ohm  G_parasitic=1e-6 1/Ohm  IL_specify=on  IL_priority=High  IL=[0, 0, 0] A  IL_nominal_specify=off  IL_nominal_value=1  IL_nominal_unit=A  VC_specify=on  VC_priority=High  VC=[0, 0, 0] V  VC_nominal_specify=off  VC_nominal_value=1  VC_nominal_unit=V
  A : PMIOPort  Side=Left
  B : PMIOPort  Port=2  Side=Left
  C : PMIOPort  Port=3  Side=Left
  a : PMIOPort  Port=4  Side=Right
  b : PMIOPort  Port=5  Side=Right
  c : PMIOPort  Port=6  Side=Right
  connections:
  Three_PhaseSeriesRLCBran/RConn3 -- c/RConn1
  Three_PhaseSeriesRLCBran/RConn2 -- b/RConn1
  Three_PhaseSeriesRLCBran/RConn1 -- a/RConn1
  C/RConn1 -- Three_PhaseSeriesRLCBran/LConn3
  B/RConn1 -- Three_PhaseSeriesRLCBran/LConn2
  A/RConn1 -- Three_PhaseSeriesRLCBran/LConn1

== system IEEE33_TR_TEMPORAL_RECOGNIZABILITY_MASTER/Three-Phase Series RLC Branch13 ==
  Three_PhaseSeriesRLCBran : ee_lib/Passive/RLC Assemblies/RLC (Three-Phase)  port_option=ee.enum.threePhasePort.expanded  component_structure=4  R=0.591 Ohm  L=0.0016743 H  C=1e-06 F  R_parasitic=1e-6 Ohm  G_parasitic=1e-6 1/Ohm  IL_specify=on  IL_priority=High  IL=[0, 0, 0] A  IL_nominal_specify=off  IL_nominal_value=1  IL_nominal_unit=A  VC_specify=on  VC_priority=High  VC=[0, 0, 0] V  VC_nominal_specify=off  VC_nominal_value=1  VC_nominal_unit=V
  A : PMIOPort  Side=Left
  B : PMIOPort  Port=2  Side=Left
  C : PMIOPort  Port=3  Side=Left
  a : PMIOPort  Port=4  Side=Right
  b : PMIOPort  Port=5  Side=Right
  c : PMIOPort  Port=6  Side=Right
  connections:
  Three_PhaseSeriesRLCBran/RConn3 -- c/RConn1
  Three_PhaseSeriesRLCBran/RConn2 -- b/RConn1
  Three_PhaseSeriesRLCBran/RConn1 -- a/RConn1
  C/RConn1 -- Three_PhaseSeriesRLCBran/LConn3
  B/RConn1 -- Three_PhaseSeriesRLCBran/LConn2
  A/RConn1 -- Three_PhaseSeriesRLCBran/LConn1

== system IEEE33_TR_TEMPORAL_RECOGNIZABILITY_MASTER/Three-Phase Series RLC Branch14 ==
  Three_PhaseSeriesRLCBran : ee_lib/Passive/RLC Assemblies/RLC (Three-Phase)  port_option=ee.enum.threePhasePort.expanded  component_structure=4  R=0.7463 Ohm  L=0.0017348 H  C=1e-06 F  R_parasitic=1e-6 Ohm  G_parasitic=1e-6 1/Ohm  IL_specify=on  IL_priority=High  IL=[0, 0, 0] A  IL_nominal_specify=off  IL_nominal_value=1  IL_nominal_unit=A  VC_specify=on  VC_priority=High  VC=[0, 0, 0] V  VC_nominal_specify=off  VC_nominal_value=1  VC_nominal_unit=V
  A : PMIOPort  Side=Left
  B : PMIOPort  Port=2  Side=Left
  C : PMIOPort  Port=3  Side=Left
  a : PMIOPort  Port=4  Side=Right
  b : PMIOPort  Port=5  Side=Right
  c : PMIOPort  Port=6  Side=Right
  connections:
  Three_PhaseSeriesRLCBran/RConn3 -- c/RConn1
  Three_PhaseSeriesRLCBran/RConn2 -- b/RConn1
  Three_PhaseSeriesRLCBran/RConn1 -- a/RConn1
  C/RConn1 -- Three_PhaseSeriesRLCBran/LConn3
  B/RConn1 -- Three_PhaseSeriesRLCBran/LConn2
  A/RConn1 -- Three_PhaseSeriesRLCBran/LConn1

== system IEEE33_TR_TEMPORAL_RECOGNIZABILITY_MASTER/Three-Phase Series RLC Branch15 ==
  Three_PhaseSeriesRLCBran : ee_lib/Passive/RLC Assemblies/RLC (Three-Phase)  port_option=ee.enum.threePhasePort.expanded  component_structure=4  R=1.289 Ohm  L=0.0054781 H  C=1e-06 F  R_parasitic=1e-6 Ohm  G_parasitic=1e-6 1/Ohm  IL_specify=on  IL_priority=High  IL=[0, 0, 0] A  IL_nominal_specify=off  IL_nominal_value=1  IL_nominal_unit=A  VC_specify=on  VC_priority=High  VC=[0, 0, 0] V  VC_nominal_specify=off  VC_nominal_value=1  VC_nominal_unit=V
  A : PMIOPort  Side=Left
  B : PMIOPort  Port=2  Side=Left
  C : PMIOPort  Port=3  Side=Left
  a : PMIOPort  Port=4  Side=Right
  b : PMIOPort  Port=5  Side=Right
  c : PMIOPort  Port=6  Side=Right
  connections:
  Three_PhaseSeriesRLCBran/RConn3 -- c/RConn1
  Three_PhaseSeriesRLCBran/RConn2 -- b/RConn1
  Three_PhaseSeriesRLCBran/RConn1 -- a/RConn1
  C/RConn1 -- Three_PhaseSeriesRLCBran/LConn3
  B/RConn1 -- Three_PhaseSeriesRLCBran/LConn2
  A/RConn1 -- Three_PhaseSeriesRLCBran/LConn1

== system IEEE33_TR_TEMPORAL_RECOGNIZABILITY_MASTER/Three-Phase Series RLC Branch16 ==
  Three_PhaseSeriesRLCBran : ee_lib/Passive/RLC Assemblies/RLC (Three-Phase)  port_option=ee.enum.threePhasePort.expanded  component_structure=4  R=0.732 Ohm  L=0.0018271 H  C=1e-06 F  R_parasitic=1e-6 Ohm  G_parasitic=1e-6 1/Ohm  IL_specify=on  IL_priority=High  IL=[0, 0, 0] A  IL_nominal_specify=off  IL_nominal_value=1  IL_nominal_unit=A  VC_specify=on  VC_priority=High  VC=[0, 0, 0] V  VC_nominal_specify=off  VC_nominal_value=1  VC_nominal_unit=V
  A : PMIOPort  Side=Left
  B : PMIOPort  Port=2  Side=Left
  C : PMIOPort  Port=3  Side=Left
  a : PMIOPort  Port=4  Side=Right
  b : PMIOPort  Port=5  Side=Right
  c : PMIOPort  Port=6  Side=Right
  connections:
  Three_PhaseSeriesRLCBran/RConn3 -- c/RConn1
  Three_PhaseSeriesRLCBran/RConn2 -- b/RConn1
  Three_PhaseSeriesRLCBran/RConn1 -- a/RConn1
  C/RConn1 -- Three_PhaseSeriesRLCBran/LConn3
  B/RConn1 -- Three_PhaseSeriesRLCBran/LConn2
  A/RConn1 -- Three_PhaseSeriesRLCBran/LConn1

== system IEEE33_TR_TEMPORAL_RECOGNIZABILITY_MASTER/Three-Phase Series RLC Branch18 ==
  Three_PhaseSeriesRLCBran : ee_lib/Passive/RLC Assemblies/RLC (Three-Phase)  port_option=ee.enum.threePhasePort.expanded  component_structure=4  R=0.164 Ohm  L=0.00049815 H  C=1e-06 F  R_parasitic=1e-6 Ohm  G_parasitic=1e-6 1/Ohm  IL_specify=on  IL_priority=High  IL=[0, 0, 0] A  IL_nominal_specify=off  IL_nominal_value=1  IL_nominal_unit=A  VC_specify=on  VC_priority=High  VC=[0, 0, 0] V  VC_nominal_specify=off  VC_nominal_value=1  VC_nominal_unit=V
  A : PMIOPort  Side=Left
  B : PMIOPort  Port=2  Side=Left
  C : PMIOPort  Port=3  Side=Left
  a : PMIOPort  Port=4  Side=Right
  b : PMIOPort  Port=5  Side=Right
  c : PMIOPort  Port=6  Side=Right
  connections:
  Three_PhaseSeriesRLCBran/RConn3 -- c/RConn1
  Three_PhaseSeriesRLCBran/RConn2 -- b/RConn1
  Three_PhaseSeriesRLCBran/RConn1 -- a/RConn1
  C/RConn1 -- Three_PhaseSeriesRLCBran/LConn3
  B/RConn1 -- Three_PhaseSeriesRLCBran/LConn2
  A/RConn1 -- Three_PhaseSeriesRLCBran/LConn1

== system IEEE33_TR_TEMPORAL_RECOGNIZABILITY_MASTER/Three-Phase Series RLC Branch19 ==
  Three_PhaseSeriesRLCBran : ee_lib/Passive/RLC Assemblies/RLC (Three-Phase)  port_option=ee.enum.threePhasePort.expanded  component_structure=4  R=1.5042 Ohm  L=0.0043144 H  C=1e-06 F  R_parasitic=1e-6 Ohm  G_parasitic=1e-6 1/Ohm  IL_specify=on  IL_priority=High  IL=[0, 0, 0] A  IL_nominal_specify=off  IL_nominal_value=1  IL_nominal_unit=A  VC_specify=on  VC_priority=High  VC=[0, 0, 0] V  VC_nominal_specify=off  VC_nominal_value=1  VC_nominal_unit=V
  A : PMIOPort  Side=Left
  B : PMIOPort  Port=2  Side=Left
  C : PMIOPort  Port=3  Side=Left
  a : PMIOPort  Port=4  Side=Right
  b : PMIOPort  Port=5  Side=Right
  c : PMIOPort  Port=6  Side=Right
  connections:
  Three_PhaseSeriesRLCBran/RConn3 -- c/RConn1
  Three_PhaseSeriesRLCBran/RConn2 -- b/RConn1
  Three_PhaseSeriesRLCBran/RConn1 -- a/RConn1
  C/RConn1 -- Three_PhaseSeriesRLCBran/LConn3
  B/RConn1 -- Three_PhaseSeriesRLCBran/LConn2
  A/RConn1 -- Three_PhaseSeriesRLCBran/LConn1

== system IEEE33_TR_TEMPORAL_RECOGNIZABILITY_MASTER/Three-Phase Series RLC Branch2 ==
  Three_PhaseSeriesRLCBran : ee_lib/Passive/RLC Assemblies/RLC (Three-Phase)  port_option=ee.enum.threePhasePort.expanded  component_structure=4  R=0.366 Ohm  L=0.00059333 H  C=1e-06 F  R_parasitic=1e-6 Ohm  G_parasitic=1e-6 1/Ohm  IL_specify=on  IL_priority=High  IL=[0, 0, 0] A  IL_nominal_specify=off  IL_nominal_value=1  IL_nominal_unit=A  VC_specify=on  VC_priority=High  VC=[0, 0, 0] V  VC_nominal_specify=off  VC_nominal_value=1  VC_nominal_unit=V
  A : PMIOPort  Side=Left
  B : PMIOPort  Port=2  Side=Left
  C : PMIOPort  Port=3  Side=Left
  a : PMIOPort  Port=4  Side=Right
  b : PMIOPort  Port=5  Side=Right
  c : PMIOPort  Port=6  Side=Right
  connections:
  Three_PhaseSeriesRLCBran/RConn3 -- c/RConn1
  Three_PhaseSeriesRLCBran/RConn2 -- b/RConn1
  Three_PhaseSeriesRLCBran/RConn1 -- a/RConn1
  C/RConn1 -- Three_PhaseSeriesRLCBran/LConn3
  B/RConn1 -- Three_PhaseSeriesRLCBran/LConn2
  A/RConn1 -- Three_PhaseSeriesRLCBran/LConn1

== system IEEE33_TR_TEMPORAL_RECOGNIZABILITY_MASTER/Three-Phase Series RLC Branch20 ==
  Three_PhaseSeriesRLCBran : ee_lib/Passive/RLC Assemblies/RLC (Three-Phase)  port_option=ee.enum.threePhasePort.expanded  component_structure=4  R=0.4095 Ohm  L=0.0015228 H  C=1e-06 F  R_parasitic=1e-6 Ohm  G_parasitic=1e-6 1/Ohm  IL_specify=on  IL_priority=High  IL=[0, 0, 0] A  IL_nominal_specify=off  IL_nominal_value=1  IL_nominal_unit=A  VC_specify=on  VC_priority=High  VC=[0, 0, 0] V  VC_nominal_specify=off  VC_nominal_value=1  VC_nominal_unit=V
  A : PMIOPort  Side=Left
  B : PMIOPort  Port=2  Side=Left
  C : PMIOPort  Port=3  Side=Left
  a : PMIOPort  Port=4  Side=Right
  b : PMIOPort  Port=5  Side=Right
  c : PMIOPort  Port=6  Side=Right
  connections:
  Three_PhaseSeriesRLCBran/RConn3 -- c/RConn1
  Three_PhaseSeriesRLCBran/RConn2 -- b/RConn1
  Three_PhaseSeriesRLCBran/RConn1 -- a/RConn1
  C/RConn1 -- Three_PhaseSeriesRLCBran/LConn3
  B/RConn1 -- Three_PhaseSeriesRLCBran/LConn2
  A/RConn1 -- Three_PhaseSeriesRLCBran/LConn1

== system IEEE33_TR_TEMPORAL_RECOGNIZABILITY_MASTER/Three-Phase Series RLC Branch21 ==
  Three_PhaseSeriesRLCBran : ee_lib/Passive/RLC Assemblies/RLC (Three-Phase)  port_option=ee.enum.threePhasePort.expanded  component_structure=4  R=0.7089 Ohm  L=0.0029835 H  C=1e-06 F  R_parasitic=1e-6 Ohm  G_parasitic=1e-6 1/Ohm  IL_specify=on  IL_priority=High  IL=[0, 0, 0] A  IL_nominal_specify=off  IL_nominal_value=1  IL_nominal_unit=A  VC_specify=on  VC_priority=High  VC=[0, 0, 0] V  VC_nominal_specify=off  VC_nominal_value=1  VC_nominal_unit=V
  A : PMIOPort  Side=Left
  B : PMIOPort  Port=2  Side=Left
  C : PMIOPort  Port=3  Side=Left
  a : PMIOPort  Port=4  Side=Right
  b : PMIOPort  Port=5  Side=Right
  c : PMIOPort  Port=6  Side=Right
  connections:
  Three_PhaseSeriesRLCBran/RConn3 -- c/RConn1
  Three_PhaseSeriesRLCBran/RConn2 -- b/RConn1
  Three_PhaseSeriesRLCBran/RConn1 -- a/RConn1
  C/RConn1 -- Three_PhaseSeriesRLCBran/LConn3
  B/RConn1 -- Three_PhaseSeriesRLCBran/LConn2
  A/RConn1 -- Three_PhaseSeriesRLCBran/LConn1

== system IEEE33_TR_TEMPORAL_RECOGNIZABILITY_MASTER/Three-Phase Series RLC Branch22 ==
  Three_PhaseSeriesRLCBran : ee_lib/Passive/RLC Assemblies/RLC (Three-Phase)  port_option=ee.enum.threePhasePort.expanded  component_structure=4  R=2 Ohm  L=0.0063662 H  C=1e-06 F  R_parasitic=1e-6 Ohm  G_parasitic=1e-6 1/Ohm  IL_specify=on  IL_priority=High  IL=[0, 0, 0] A  IL_nominal_specify=off  IL_nominal_value=1  IL_nominal_unit=A  VC_specify=on  VC_priority=High  VC=[0, 0, 0] V  VC_nominal_specify=off  VC_nominal_value=1  VC_nominal_unit=V
  A : PMIOPort  Side=Left
  B : PMIOPort  Port=2  Side=Left
  C : PMIOPort  Port=3  Side=Left
  a : PMIOPort  Port=4  Side=Right
  b : PMIOPort  Port=5  Side=Right
  c : PMIOPort  Port=6  Side=Right
  connections:
  Three_PhaseSeriesRLCBran/RConn3 -- c/RConn1
  Three_PhaseSeriesRLCBran/RConn2 -- b/RConn1
  Three_PhaseSeriesRLCBran/RConn1 -- a/RConn1
  C/RConn1 -- Three_PhaseSeriesRLCBran/LConn3
  B/RConn1 -- Three_PhaseSeriesRLCBran/LConn2
  A/RConn1 -- Three_PhaseSeriesRLCBran/LConn1

== system IEEE33_TR_TEMPORAL_RECOGNIZABILITY_MASTER/Three-Phase Series RLC Branch23 ==
  Three_PhaseSeriesRLCBran : ee_lib/Passive/RLC Assemblies/RLC (Three-Phase)  port_option=ee.enum.threePhasePort.expanded  component_structure=4  R=0.4512 Ohm  L=0.00098135 H  C=1e-06 F  R_parasitic=1e-6 Ohm  G_parasitic=1e-6 1/Ohm  IL_specify=on  IL_priority=High  IL=[0, 0, 0] A  IL_nominal_specify=off  IL_nominal_value=1  IL_nominal_unit=A  VC_specify=on  VC_priority=High  VC=[0, 0, 0] V  VC_nominal_specify=off  VC_nominal_value=1  VC_nominal_unit=V
  A : PMIOPort  Side=Left
  B : PMIOPort  Port=2  Side=Left
  C : PMIOPort  Port=3  Side=Left
  a : PMIOPort  Port=4  Side=Right
  b : PMIOPort  Port=5  Side=Right
  c : PMIOPort  Port=6  Side=Right
  connections:
  Three_PhaseSeriesRLCBran/RConn3 -- c/RConn1
  Three_PhaseSeriesRLCBran/RConn2 -- b/RConn1
  Three_PhaseSeriesRLCBran/RConn1 -- a/RConn1
  C/RConn1 -- Three_PhaseSeriesRLCBran/LConn3
  B/RConn1 -- Three_PhaseSeriesRLCBran/LConn2
  A/RConn1 -- Three_PhaseSeriesRLCBran/LConn1

== system IEEE33_TR_TEMPORAL_RECOGNIZABILITY_MASTER/Three-Phase Series RLC Branch24 ==
  Three_PhaseSeriesRLCBran : ee_lib/Passive/RLC Assemblies/RLC (Three-Phase)  port_option=ee.enum.threePhasePort.expanded  component_structure=4  R=0.898 Ohm  L=0.0022571 H  C=1e-06 F  R_parasitic=1e-6 Ohm  G_parasitic=1e-6 1/Ohm  IL_specify=on  IL_priority=High  IL=[0, 0, 0] A  IL_nominal_specify=off  IL_nominal_value=1  IL_nominal_unit=A  VC_specify=on  VC_priority=High  VC=[0, 0, 0] V  VC_nominal_specify=off  VC_nominal_value=1  VC_nominal_unit=V
  A : PMIOPort  Side=Left
  B : PMIOPort  Port=2  Side=Left
  C : PMIOPort  Port=3  Side=Left
  a : PMIOPort  Port=4  Side=Right
  b : PMIOPort  Port=5  Side=Right
  c : PMIOPort  Port=6  Side=Right
  connections:
  Three_PhaseSeriesRLCBran/RConn3 -- c/RConn1
  Three_PhaseSeriesRLCBran/RConn2 -- b/RConn1
  Three_PhaseSeriesRLCBran/RConn1 -- a/RConn1
  C/RConn1 -- Three_PhaseSeriesRLCBran/LConn3
  B/RConn1 -- Three_PhaseSeriesRLCBran/LConn2
  A/RConn1 -- Three_PhaseSeriesRLCBran/LConn1

== system IEEE33_TR_TEMPORAL_RECOGNIZABILITY_MASTER/Three-Phase Series RLC Branch25 ==
  Three_PhaseSeriesRLCBran : ee_lib/Passive/RLC Assemblies/RLC (Three-Phase)  port_option=ee.enum.threePhasePort.expanded  component_structure=4  R=0.896 Ohm  L=0.0022317 H  C=1e-06 F  R_parasitic=1e-6 Ohm  G_parasitic=1e-6 1/Ohm  IL_specify=on  IL_priority=High  IL=[0, 0, 0] A  IL_nominal_specify=off  IL_nominal_value=1  IL_nominal_unit=A  VC_specify=on  VC_priority=High  VC=[0, 0, 0] V  VC_nominal_specify=off  VC_nominal_value=1  VC_nominal_unit=V
  A : PMIOPort  Side=Left
  B : PMIOPort  Port=2  Side=Left
  C : PMIOPort  Port=3  Side=Left
  a : PMIOPort  Port=4  Side=Right
  b : PMIOPort  Port=5  Side=Right
  c : PMIOPort  Port=6  Side=Right
  connections:
  Three_PhaseSeriesRLCBran/RConn3 -- c/RConn1
  Three_PhaseSeriesRLCBran/RConn2 -- b/RConn1
  Three_PhaseSeriesRLCBran/RConn1 -- a/RConn1
  C/RConn1 -- Three_PhaseSeriesRLCBran/LConn3
  B/RConn1 -- Three_PhaseSeriesRLCBran/LConn2
  A/RConn1 -- Three_PhaseSeriesRLCBran/LConn1

== system IEEE33_TR_TEMPORAL_RECOGNIZABILITY_MASTER/Three-Phase Series RLC Branch27 ==
  Three_PhaseSeriesRLCBran : ee_lib/Passive/RLC Assemblies/RLC (Three-Phase)  port_option=ee.enum.threePhasePort.expanded  component_structure=4  R=0.203 Ohm  L=0.00032913 H  C=1e-06 F  R_parasitic=1e-6 Ohm  G_parasitic=1e-6 1/Ohm  IL_specify=on  IL_priority=High  IL=[0, 0, 0] A  IL_nominal_specify=off  IL_nominal_value=1  IL_nominal_unit=A  VC_specify=on  VC_priority=High  VC=[0, 0, 0] V  VC_nominal_specify=off  VC_nominal_value=1  VC_nominal_unit=V
  A : PMIOPort  Side=Left
  B : PMIOPort  Port=2  Side=Left
  C : PMIOPort  Port=3  Side=Left
  a : PMIOPort  Port=4  Side=Right
  b : PMIOPort  Port=5  Side=Right
  c : PMIOPort  Port=6  Side=Right
  connections:
  Three_PhaseSeriesRLCBran/RConn3 -- c/RConn1
  Three_PhaseSeriesRLCBran/RConn2 -- b/RConn1
  Three_PhaseSeriesRLCBran/RConn1 -- a/RConn1
  C/RConn1 -- Three_PhaseSeriesRLCBran/LConn3
  B/RConn1 -- Three_PhaseSeriesRLCBran/LConn2
  A/RConn1 -- Three_PhaseSeriesRLCBran/LConn1

== system IEEE33_TR_TEMPORAL_RECOGNIZABILITY_MASTER/Three-Phase Series RLC Branch28 ==
  Three_PhaseSeriesRLCBran : ee_lib/Passive/RLC Assemblies/RLC (Three-Phase)  port_option=ee.enum.threePhasePort.expanded  component_structure=4  R=0.2842 Ohm  L=0.00046059 H  C=1e-06 F  R_parasitic=1e-6 Ohm  G_parasitic=1e-6 1/Ohm  IL_specify=on  IL_priority=High  IL=[0, 0, 0] A  IL_nominal_specify=off  IL_nominal_value=1  IL_nominal_unit=A  VC_specify=on  VC_priority=High  VC=[0, 0, 0] V  VC_nominal_specify=off  VC_nominal_value=1  VC_nominal_unit=V
  A : PMIOPort  Side=Left
  B : PMIOPort  Port=2  Side=Left
  C : PMIOPort  Port=3  Side=Left
  a : PMIOPort  Port=4  Side=Right
  b : PMIOPort  Port=5  Side=Right
  c : PMIOPort  Port=6  Side=Right
  connections:
  Three_PhaseSeriesRLCBran/RConn3 -- c/RConn1
  Three_PhaseSeriesRLCBran/RConn2 -- b/RConn1
  Three_PhaseSeriesRLCBran/RConn1 -- a/RConn1
  C/RConn1 -- Three_PhaseSeriesRLCBran/LConn3
  B/RConn1 -- Three_PhaseSeriesRLCBran/LConn2
  A/RConn1 -- Three_PhaseSeriesRLCBran/LConn1

== system IEEE33_TR_TEMPORAL_RECOGNIZABILITY_MASTER/Three-Phase Series RLC Branch29 ==
  Three_PhaseSeriesRLCBran : ee_lib/Passive/RLC Assemblies/RLC (Three-Phase)  port_option=ee.enum.threePhasePort.expanded  component_structure=4  R=1.059 Ohm  L=0.0029721 H  C=1e-06 F  R_parasitic=1e-6 Ohm  G_parasitic=1e-6 1/Ohm  IL_specify=on  IL_priority=High  IL=[0, 0, 0] A  IL_nominal_specify=off  IL_nominal_value=1  IL_nominal_unit=A  VC_specify=on  VC_priority=High  VC=[0, 0, 0] V  VC_nominal_specify=off  VC_nominal_value=1  VC_nominal_unit=V
  A : PMIOPort  Side=Left
  B : PMIOPort  Port=2  Side=Left
  C : PMIOPort  Port=3  Side=Left
  a : PMIOPort  Port=4  Side=Right
  b : PMIOPort  Port=5  Side=Right
  c : PMIOPort  Port=6  Side=Right
  connections:
  Three_PhaseSeriesRLCBran/RConn3 -- c/RConn1
  Three_PhaseSeriesRLCBran/RConn2 -- b/RConn1
  Three_PhaseSeriesRLCBran/RConn1 -- a/RConn1
  C/RConn1 -- Three_PhaseSeriesRLCBran/LConn3
  B/RConn1 -- Three_PhaseSeriesRLCBran/LConn2
  A/RConn1 -- Three_PhaseSeriesRLCBran/LConn1

== system IEEE33_TR_TEMPORAL_RECOGNIZABILITY_MASTER/Three-Phase Series RLC Branch3 ==
  Three_PhaseSeriesRLCBran : ee_lib/Passive/RLC Assemblies/RLC (Three-Phase)  port_option=ee.enum.threePhasePort.expanded  component_structure=4  R=0.3811 Ohm  L=0.00061784 H  C=1e-06 F  R_parasitic=1e-6 Ohm  G_parasitic=1e-6 1/Ohm  IL_specify=on  IL_priority=High  IL=[0, 0, 0] A  IL_nominal_specify=off  IL_nominal_value=1  IL_nominal_unit=A  VC_specify=on  VC_priority=High  VC=[0, 0, 0] V  VC_nominal_specify=off  VC_nominal_value=1  VC_nominal_unit=V
  A : PMIOPort  Side=Left
  B : PMIOPort  Port=2  Side=Left
  C : PMIOPort  Port=3  Side=Left
  a : PMIOPort  Port=4  Side=Right
  b : PMIOPort  Port=5  Side=Right
  c : PMIOPort  Port=6  Side=Right
  connections:
  Three_PhaseSeriesRLCBran/RConn3 -- c/RConn1
  Three_PhaseSeriesRLCBran/RConn2 -- b/RConn1
  Three_PhaseSeriesRLCBran/RConn1 -- a/RConn1
  C/RConn1 -- Three_PhaseSeriesRLCBran/LConn3
  B/RConn1 -- Three_PhaseSeriesRLCBran/LConn2
  A/RConn1 -- Three_PhaseSeriesRLCBran/LConn1

== system IEEE33_TR_TEMPORAL_RECOGNIZABILITY_MASTER/Three-Phase Series RLC Branch30 ==
  Three_PhaseSeriesRLCBran : ee_lib/Passive/RLC Assemblies/RLC (Three-Phase)  port_option=ee.enum.threePhasePort.expanded  component_structure=4  R=0.8042 Ohm  L=0.0022301 H  C=1e-06 F  R_parasitic=1e-6 Ohm  G_parasitic=1e-6 1/Ohm  IL_specify=on  IL_priority=High  IL=[0, 0, 0] A  IL_nominal_specify=off  IL_nominal_value=1  IL_nominal_unit=A  VC_specify=on  VC_priority=High  VC=[0, 0, 0] V  VC_nominal_specify=off  VC_nominal_value=1  VC_nominal_unit=V
  A : PMIOPort  Side=Left
  B : PMIOPort  Port=2  Side=Left
  C : PMIOPort  Port=3  Side=Left
  a : PMIOPort  Port=4  Side=Right
  b : PMIOPort  Port=5  Side=Right
  c : PMIOPort  Port=6  Side=Right
  connections:
  Three_PhaseSeriesRLCBran/RConn3 -- c/RConn1
  Three_PhaseSeriesRLCBran/RConn2 -- b/RConn1
  Three_PhaseSeriesRLCBran/RConn1 -- a/RConn1
  C/RConn1 -- Three_PhaseSeriesRLCBran/LConn3
  B/RConn1 -- Three_PhaseSeriesRLCBran/LConn2
  A/RConn1 -- Three_PhaseSeriesRLCBran/LConn1
